simulink model "mcb_pmsm_fsfb_qep_f28379d"  (R2025b)
settings: Solver=FixedStepDiscrete  StartTime=0.0  StopTime=4  RelTol=1e-3  EnableMultiTasking=on
InitFcn:
  | mcb_pmsm_foc_qep_f28379d_SIUnit_data;
values from neighbouring files (symbols this model uses):
  A = [ -Rs/L,           0,                  0 ... (first row only)    [mcb_pmsm_fsfb_f28379d_param.m]    (also in v0_pmsm_fsfb_sim_for_flipsky_.m = [; v1_0_3_sim_param_fsfc.m = [)
  dataType = 'single'    [mcb_pmsm_foc_qep_f28379d_SIUnit_data.m]
  inverter = mcb.updateInverterParameters(pmsm,inverter,target)    [mcb_pmsm_foc_qep_f28379d_SIUnit_data.m]
  lambda_pm = pmsm.FluxPM    [mcb_pmsm_foc_qep_f28379d_SIUnit_data.m]
  PI_params = mcb.calcFOCGains(motor,Ts,Ts_speed,SpdLPFltCoeff=LPFltCoeff)    [mcb_pmsm_foc_qep_f28379d_SIUnit_data.m]
  pmsm = mcb.getPMSMParameters('Teknic2310P')    [mcb_pmsm_foc_qep_f28379d_SIUnit_data.m]
  T_pwm = 1/PWM_frequency    (= 5e-05)    [mcb_pmsm_foc_qep_f28379d_SIUnit_data.m]
  target = mcb.getProcessorParameters('F28379D',PWM_frequency)    [mcb_pmsm_foc_qep_f28379d_SIUnit_data.m]
  Ts = T_pwm    (= 5e-05)    [mcb_pmsm_foc_qep_f28379d_SIUnit_data.m]    (also in v0_pmsm_fsfb_sim_for_flipsky_.m = 0.0001; v1_0_3_sim_param_fsfc.m = 0.0001)
  Ts_inverter = T_pwm/2    (= 2.5e-05)    [mcb_pmsm_foc_qep_f28379d_SIUnit_data.m]
  Ts_motor = T_pwm/2    (= 2.5e-05)    [mcb_pmsm_foc_qep_f28379d_SIUnit_data.m]
  Ts_simulink = T_pwm/2    (= 2.5e-05)    [mcb_pmsm_foc_qep_f28379d_SIUnit_data.m]
  Ts_speed = 10*Ts    (= 0.0005)    [mcb_pmsm_foc_qep_f28379d_SIUnit_data.m]
undefined symbols (not defined in the file or in its folder): bit, DiscIntNeverNeededParam, Down, GPTRIP1SEL, GPTRIP2SEL, TZ1, TZ2, Up
libraries: mcbcontrolslib x8, c2802xlib x7, simulink x7, c280xlib x5, c2837xDlib x4, mcbeeMathTransformLib x3, slpidlib x3, mcbpositiondecoderlib x3, c2000lib x1, svdutilitieslib x1, autolibpmsmexterior x1
(part 1 of 2)
settings Model: ExtModeTrigDuration=8  Creator=The MathWorks, Inc.  LastModifiedBy=LabPC
settings SolverCC: AlgebraicLoopSolver=TrustRegion
settings OptimizationCC: DefaultParameterBehavior=Inlined  DefaultUnderspecifiedDataType=single  EnhancedBackFolding=on  PassReuseOutputArgsAs=Individual arguments  MaxStackSize=1024  OptimizeBlockOrder=speed  DifferentSizesBufferReuse=on  OptimizationCustomize=off  DenormalBehavior=FlushToZero  EfficientTunableParamExpr=on
settings DebuggingCC: MultiTaskDSMMsg=none  IntegerOverflowMsg=none  ParameterPrecisionLossMsg=none  ParameterTunabilityLossMsg=error  UnconnectedInputMsg=warning  UnconnectedOutputMsg=warning  UnconnectedLineMsg=warning
settings HardwareCC: ProdBitPerChar=16.0  ProdBitPerInt=16.0  ProdBitPerPointer=32.0  ProdBitPerSizeT=32.0  ProdBitPerPtrDiffT=32.0  ProdLargestAtomicInteger=Integer  ProdLargestAtomicFloat=None  ProdWordSize=16.0  ProdLongLongMode=on  ProdHWDeviceType=Texas Instruments->C2000
settings ModelReferenceCC: EnableRefExpFcnMdlSchedulingChecks=on
settings SFSimCC: MATLABDynamicMemAlloc=off
settings RTWCC: SystemTargetFile=ert.tlc  HardwareBoard=TI Delfino F28379D LaunchPad  TemplateMakefile=ert_default_tmf  Toolchain=Texas Instruments Code Composer Studio (C2000)  GPUComputeCapability=3.5  DLArmComputeVersion=19.05  Description=Embedded Coder
settings CodeAppCC: ForceParamTrailComments=on  IgnoreCustomStorageClasses=off  OperatorAnnotations=on  SimulinkDataObjDesc=on  SFDataObjDesc=on  InsertBlockDesc=on
settings ERTTargetCC: ExtModeStaticAllocSize=10000.0  InlinedParameterPlacement=Hierarchical  MemSecPackage=tic2000demospkg  DynamicArrayContainerType=coder::array  CodeReplacementLibrary=TI C28x

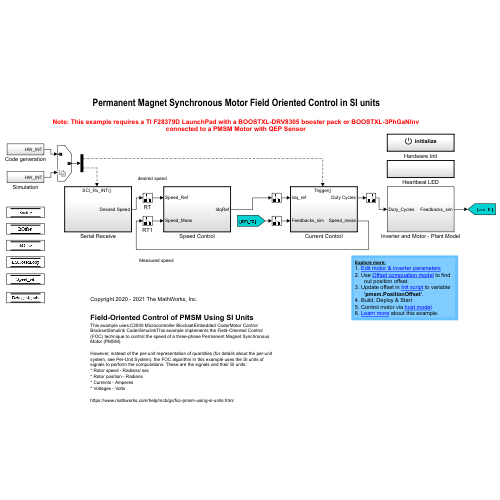
[thumbnail: Simulink's stored preview of the top-level diagram]
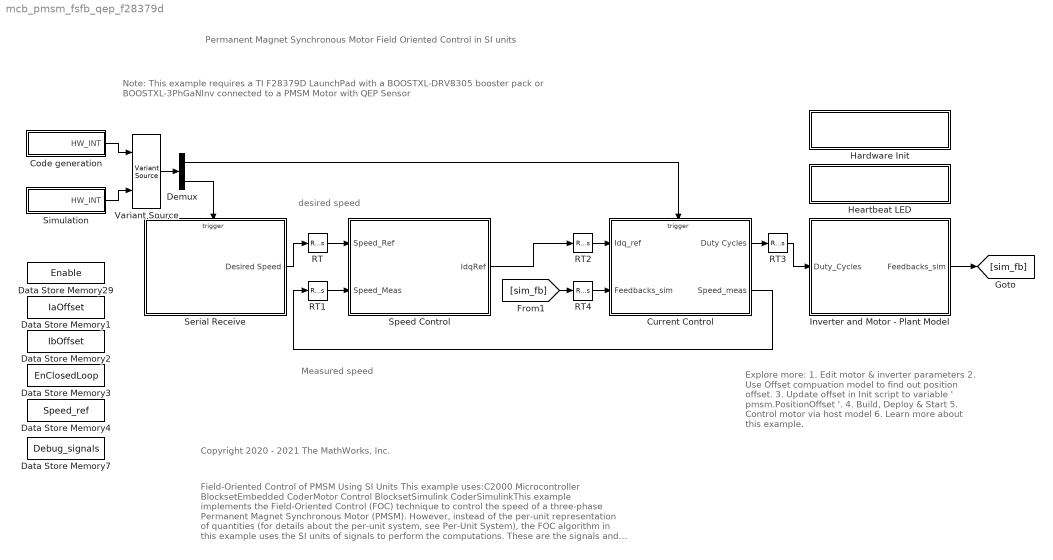
== system mcb_pmsm_fsfb_qep_f28379d ==
  note: Measured speed
  note: Field-Oriented Control of PMSM Using SI Units
      | This example uses:C2000 Microcontroller BlocksetEmbedded CoderMotor Control BlocksetSimulink CoderSimulinkThis example implements the Field-Oriented Control (FOC) technique to control the speed of a three-phase Permanent Magnet Synchronous Motor (PMSM).
      |
      | However, instead of the per-unit representation of quantities (for details about the per-unit system, see Per-Unit System), the FOC algorithm in this example uses the SI units of signals to perform the computations. These are the signals and their SI units:
      | * Rotor speed - Radians/ sec
      | * Rotor position - Radians
      | * Currents - Amperes
      | * Voltages - Volts
      |
      | https://www.mathworks.com/help/mcb/gs/foc-pmsm-using-si-units.html
  note: Permanent Magnet Synchronous Motor Field Oriented Control in SI units
  note: Copyright 2020 - 2021 The MathWorks, Inc.
  note: Note: This example requires a TI F28379D LaunchPad with a BOOSTXL-DRV8305 booster pack or BOOSTXL-3PhGaNInv
      | connected to a PMSM Motor with QEP Sensor
  note: Explore more:
      | 1. Edit motor & inverter parameters
      | 2. Use Offset compuation model to find out position offset.
      | 3. Update offset in Init script to variable ' pmsm.PositionOffset '.
      | 4. Build, Deploy & Start
      | 5. Control motor via host model
      | 6. Learn more about this example.
  note: desired speed
  Code generation : Subsystem
  Current Control : Subsystem
      settings: RTWSystemCode=Nonreusable function
  Data Store Memory1 : DataStoreMemory  DataStoreName=IaOffset  InitialValue=inverter.CtSensAOffset  ShowAdditionalParam=off
  Data Store Memory2 : DataStoreMemory  DataStoreName=IbOffset  InitialValue=inverter.CtSensBOffset  ShowAdditionalParam=off
  Data Store Memory29 : DataStoreMemory  DataStoreName=Enable  ShowAdditionalParam=off  OutDataTypeStr=boolean
  Data Store Memory3 : DataStoreMemory  DataStoreName=EnClosedLoop  ShowAdditionalParam=off  OutDataTypeStr=boolean
  Data Store Memory4 : DataStoreMemory  DataStoreName=Speed_ref  ShowAdditionalParam=off  OutDataTypeStr=dataType
  Data Store Memory7 : DataStoreMemory  DataStoreName=Debug_signals  InitialValue=5  ShowAdditionalParam=off  OutDataTypeStr=uint16
  Demux : Demux  Outputs=2
  Hardware Init : Subsystem  TreatAsAtomicUnit=on
  Heartbeat LED : Subsystem  TreatAsAtomicUnit=on
  Inverter and Motor - Plant Model : Subsystem
  RT : RateTransition  Deterministic=off  OutPortSampleTime=Ts_speed
  RT1 : RateTransition  Deterministic=off  OutPortSampleTime=Ts_speed
  RT2 : RateTransition  Deterministic=off
  RT3 : RateTransition  Deterministic=off
  RT4 : RateTransition  Deterministic=off
  Serial Receive : Subsystem  SystemSampleTime=1e-3
  Simulation : Subsystem
  Speed Control : Subsystem  TreatAsAtomicUnit=on  SystemSampleTime=Ts_speed
  Variant Source : VariantSource  VariantControlMode=sim codegen switching  VariantControls={(codegen), (sim)}
  wires:
  Speed Control/1(IdqRef) -> RT2/1
  Demux/2 -> Serial Receive/Trigger
  RT1/1 -> Speed Control/2(Speed_Meas)
  Serial Receive/1(Desired Speed) -> RT/1
  Code generation/1(HW_INT) -> Variant Source/1
  RT4/1 -> Current Control/2(Feedbacks_sim)
  Variant Source/1 -> Demux/1
  Current Control/1(Duty Cycles) -> RT3/1
  RT/1 -> Speed Control/1(Speed_Ref)
  Demux/1 -> Current Control/Trigger
  Simulation/1(HW_INT) -> Variant Source/2
  RT3/1 -> Inverter and Motor - Plant Model/1(Duty_Cycles)
  [sim_fb] -> RT4/1
  Current Control/2(Speed_meas) -> RT1/1
  Inverter and Motor - Plant Model/1(Feedbacks_sim) -> [sim_fb]
  RT2/1 -> Current Control/1(Idq_ref)

== system mcb_pmsm_fsfb_qep_f28379d/Code generation ==
  C28x Hardware Interrupt : c2000lib/Scheduling/C28x Hardware Interrupt  irqnumbers=[1 9]  pienumbers=[2 1]  irqpriorities=[30 50]  irqpreempts=[1 0]  showinput=off  dspchiptype=C280X
  HW_INT : Outport
  wires:
  C28x Hardware Interrupt/1 -> HW_INT/1

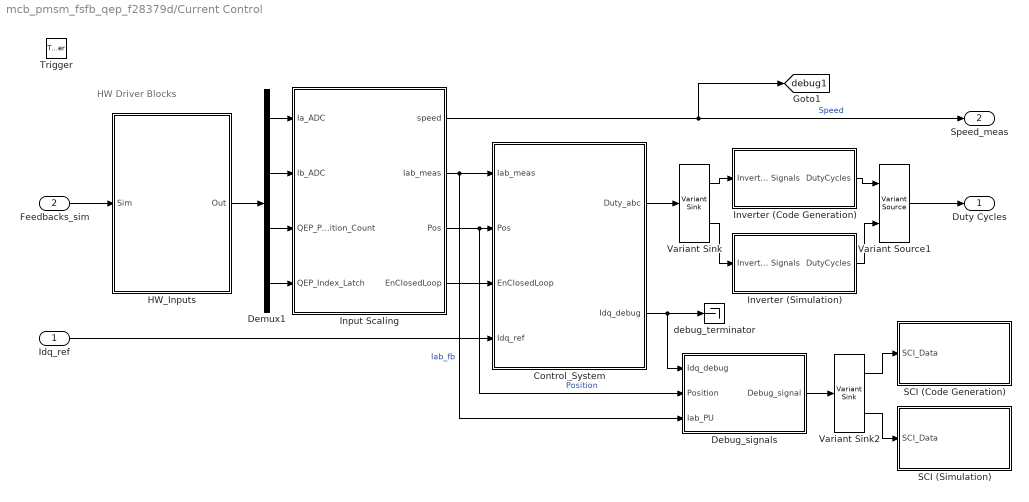
== system mcb_pmsm_fsfb_qep_f28379d/Current Control ==
  note: HW Driver Blocks
  Idq_ref : Inport
  Feedbacks_sim : Inport  Port=2
  Trigger : TriggerPort  TriggerType=function-call  VariantControl=Variant  PortDimensions=1
  Control_System : Subsystem  TreatAsAtomicUnit=on
  Debug_signals : Subsystem
  Demux1 : Demux
  HW_Inputs : Subsystem  Variant=on  VariantControlMode=sim codegen switching
  Input Scaling : Subsystem
  Inverter (Code Generation) : Subsystem
  Inverter (Simulation) : Subsystem
  SCI (Code Generation) : Subsystem
  SCI (Simulation) : Subsystem
  Variant Sink : VariantSink  VariantControlMode=sim codegen switching  VariantControls={(codegen), (sim)}
  Variant Sink2 : VariantSink  VariantControlMode=sim codegen switching  VariantControls={(codegen), (sim)}
  Variant Source1 : VariantSource  VariantControlMode=sim codegen switching  VariantControls={(codegen), (sim)}
  debug_terminator : Terminator
  Duty Cycles : Outport  InitialOutput=0  VectorParamsAs1DForOutWhenUnconnected=off
  Speed_meas : Outport  Port=2  InitialOutput=0  VectorParamsAs1DForOutWhenUnconnected=off
  tag scope: debug1=global
  wires:
  Control_System/1(Duty_abc) -> Variant Sink/1
  Input Scaling/3(Pos) -> Debug_signals/2(Position), Control_System/2(Pos)  "Position"
  Idq_ref/1 -> Control_System/4(Idq_ref)
  Input Scaling/1(speed) -> [debug1], Speed_meas/1  "Speed"
  Input Scaling/2(Iab_meas) -> Debug_signals/3(Iab_PU), Control_System/1(Iab_meas)  "Iab_fb"
  Demux1/1 -> Input Scaling/1(Ia_ADC)
  Demux1/2 -> Input Scaling/2(Ib_ADC)
  Demux1/3 -> Input Scaling/3(QEP_Position_Count)
  Demux1/4 -> Input Scaling/4(QEP_Index_Latch)
  Variant Sink2/1 -> SCI (Code Generation)/1(SCI_Data)
  Debug_signals/1(Debug_signal) -> Variant Sink2/1
  Inverter (Simulation)/1(DutyCycles) -> Variant Source1/2
  Inverter (Code Generation)/1(DutyCycles) -> Variant Source1/1
  Variant Sink2/2 -> SCI (Simulation)/1(SCI_Data)
  Variant Sink/2 -> Inverter (Simulation)/1(Inverter Signals)
  Variant Sink/1 -> Inverter (Code Generation)/1(Inverter Signals)
  Variant Source1/1 -> Duty Cycles/1
  HW_Inputs/1(Out) -> Demux1/1
  Feedbacks_sim/1 -> HW_Inputs/1(Sim)
  Control_System/2(Idq_debug) -> Debug_signals/1(Idq_debug), debug_terminator/1
  Input Scaling/4(EnClosedLoop) -> Control_System/3(EnClosedLoop)

== system mcb_pmsm_fsfb_qep_f28379d/Hardware Init ==
  6PWM_Mode : Constant  Priority=1000  Value=0x3A16  OutDataTypeStr=uint16  SampleTime=-1
  ADC_Gain_Setting : Constant  Priority=1000  Value=inverter.SPI_Gain_Setting  OutDataTypeStr=uint16  SampleTime=-1
  Code Generation : Subsystem
  Event Listener : EventListener  DisableCoverage=on  EventName=reset
  Mux : Mux  Inputs=2
  Simulation : Subsystem
  Variant Sink : VariantSink  VariantControlMode=sim codegen switching  VariantControls={(codegen), (sim)}
  wires:
  6PWM_Mode/1 -> Mux/1
  ADC_Gain_Setting/1 -> Mux/2
  Mux/1 -> Variant Sink/1
  Variant Sink/1 -> Code Generation/1(In)
  Variant Sink/2 -> Simulation/1(In1)

== system mcb_pmsm_fsfb_qep_f28379d/Heartbeat LED ==
  note: Heartbeat LED 1HZ
  Code generation : Subsystem
  RED_LED : Constant  OutDataTypeStr=uint16  SampleTime=0.5
  Simulation : Subsystem
  Variant Sink : VariantSink  VariantControlMode=sim codegen switching  VariantControls={(codegen), (sim)}
  wires:
  RED_LED/1 -> Variant Sink/1
  Variant Sink/1 -> Code generation/1(In1)
  Variant Sink/2 -> Simulation/1(In1)

== system mcb_pmsm_fsfb_qep_f28379d/Inverter and Motor - Plant Model ==
  Duty_Cycles : Inport
  Codegeneration : Subsystem
  Simulation : Subsystem
  Variant Sink : VariantSink  VariantControlMode=sim codegen switching  VariantControls={(codegen), (sim)}
  Variant Source1 : VariantSource  VariantControlMode=sim codegen switching  VariantControls={(codegen), (sim)}
  Feedbacks_sim : Outport  VectorParamsAs1DForOutWhenUnconnected=off
  wires:
  Variant Source1/1 -> Feedbacks_sim/1
  Simulation/1(Feedbacks) -> Variant Source1/2
  Codegeneration/1(Feedbacks) -> Variant Source1/1
  Duty_Cycles/1 -> Variant Sink/1
  Variant Sink/2 -> Simulation/1(Duty_Cycles)
  Variant Sink/1 -> Codegeneration/1(Duty_Cycles)

== system mcb_pmsm_fsfb_qep_f28379d/Serial Receive ==
  SCI_Rx_INT : TriggerPort  TriggerType=function-call  VariantControl=Variant
  Code Generation : Subsystem
  Data Store Write : DataStoreWrite  DataStoreName=Enable  IndexOptions=Index vector (dialog)  Indices=1  OutputSizes=1
  Data Store Write1 : DataStoreWrite  DataStoreName=Speed_ref  IndexOptions=Index vector (dialog)  Indices=1  OutputSizes=1
  Data Store Write2 : DataStoreWrite  DataStoreName=Debug_signals  IndexOptions=Index vector (dialog)  Indices=1  OutputSizes=1
  Data_Conditioning_Rx : Subsystem  Variant=on
  Simulation : Subsystem
  Variant Source : VariantSource  VariantControlMode=sim codegen switching  VariantControls={(codegen), (sim)}
  unParse : Subsystem
  Desired Speed : Outport  VectorParamsAs1DForOutWhenUnconnected=off
  wires:
  Simulation/1(Data) -> Variant Source/2
  Variant Source/1 -> Data_Conditioning_Rx/1(In1)
  Code Generation/1(Data) -> Variant Source/1
  unParse/1(Enable_PWM) -> Data Store Write/1
  Data_Conditioning_Rx/1(Desired Speed) -> Data Store Write1/1, Desired Speed/1
  Data_Conditioning_Rx/2(Out2) -> unParse/1(Data)
  unParse/2(Debug_signals) -> Data Store Write2/1

== system mcb_pmsm_fsfb_qep_f28379d/Simulation ==
  ADCINT1 : FunctionCallGenerator  SampleTime=Ts
  Mux : Mux  Inputs=2
  SCI_Rx_INT : FunctionCallGenerator  SampleTime=0.1
  HW_INT : Outport
  wires:
  SCI_Rx_INT/1 -> Mux/2
  ADCINT1/1 -> Mux/1
  Mux/1 -> HW_INT/1

== system mcb_pmsm_fsfb_qep_f28379d/Speed Control ==
  Speed_Ref : Inport
  Speed_Meas : Inport  Port=2
  Id_ref : Constant  Value=0  OutDataTypeStr=dataType  SampleTime=Ts_speed
  Mux1 : Mux  Inputs=2
  PI_Controller_Speed : Subsystem
  Subsystem : Subsystem
  IdqRef : Outport  VectorParamsAs1DForOutWhenUnconnected=off
  wires:
  Speed_Meas/1 -> PI_Controller_Speed/2(N_fb), Subsystem/2(Speed_Ref_Open)  "Speed_fb"
  Subsystem/1(Speed_Ref_PU) -> PI_Controller_Speed/1(N_ref)  "Speed_Ref"
  Id_ref/1 -> Mux1/1
  PI_Controller_Speed/1(Iq_ref) -> Mux1/2
  Mux1/1 -> IdqRef/1
  Speed_Ref/1 -> Subsystem/1(Speed_Ref_In)

== system mcb_pmsm_fsfb_qep_f28379d/Current Control/Control_System ==
  Iab_meas : Inport
  Pos : Inport  Port=2
  EnClosedLoop : Inport  Port=3
  Idq_ref : Inport  Port=4
  Closed Loop Control : Subsystem
  NOT : Logic  Operator=NOT  IconShape=distinctive  AllPortsSameDT=off  OutDataTypeStr=boolean
  Open Loop Start-Up : Subsystem
  Switch4 : Switch  Threshold=0.5  OutDataTypeStr=Inherit: Inherit via back propagation  RndMeth=Simplest  SaturateOnIntegerOverflow=off  InputSameDT=off
  Duty_abc : Outport  VectorParamsAs1DForOutWhenUnconnected=off
  Idq_debug : Outport  Port=2  VectorParamsAs1DForOutWhenUnconnected=off
  wires:
  EnClosedLoop/1 -> NOT/1, Switch4/2, Closed Loop Control/Enable
  Open Loop Start-Up/1(Duty_abc) -> Switch4/3
  Iab_meas/1 -> Closed Loop Control/1(Iab_meas)
  Pos/1 -> Closed Loop Control/2(Pos)
  Idq_ref/1 -> Closed Loop Control/3(Idq_ref)
  Closed Loop Control/2(Duty_abc) -> Switch4/1
  NOT/1 -> Open Loop Start-Up/Enable
  Switch4/1 -> Duty_abc/1  "PWM_Duty_Cycles"
  Closed Loop Control/1(Idq_debug) -> Idq_debug/1

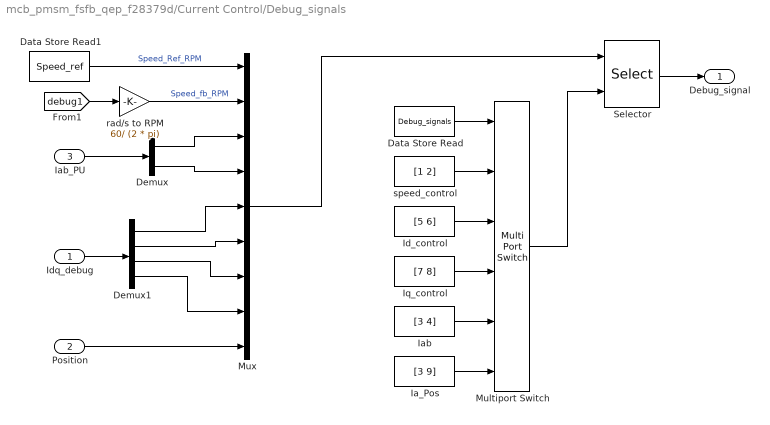
== system mcb_pmsm_fsfb_qep_f28379d/Current Control/Debug_signals ==
  Idq_debug : Inport
  Position : Inport  Port=2
  Iab_PU : Inport  Port=3
  Data Store Read : DataStoreRead  DataStoreName=Debug_signals  IndexOptions=Index vector (dialog)  Indices=1  OutputSizes=1
  Data Store Read1 : DataStoreRead  DataStoreName=Speed_ref  IndexOptions=Index vector (dialog)  Indices=1  OutputSizes=1
  Demux : Demux  Outputs=2
  Demux1 : Demux
  Ia_Pos : Constant  Value=[3 9]  OutDataTypeStr=uint16  SampleTime=-1
  Iab : Constant  Value=[3 4]  OutDataTypeStr=uint16  SampleTime=-1
  Id_control : Constant  Value=[5 6]  OutDataTypeStr=uint16  SampleTime=-1
  Iq_control : Constant  Value=[7 8]  OutDataTypeStr=uint16  SampleTime=-1
  Multiport Switch : MultiPortSwitch  Inputs=5  DiagnosticForDefault=Warning  OutDataTypeStr=uint16  RndMeth=Simplest  SaturateOnIntegerOverflow=off  InputSameDT=off
  Mux : Mux  Inputs=9
  Selector : Selector  InputPortWidth=9  IndexOptions=Index vector (port)  Indices=[1 3]  OutputSizes=1
  rad/s to RPM : Gain  Gain=60/ (2 * pi)  RndMeth=Simplest  OutDataTypeStr=Inherit: Same as input
  speed_control : Constant  Value=[1 2]  OutDataTypeStr=uint16  SampleTime=-1
  Debug_signal : Outport
  wires:
  speed_control/1 -> Multiport Switch/2
  Id_control/1 -> Multiport Switch/3
  Iq_control/1 -> Multiport Switch/4
  Iab/1 -> Multiport Switch/5
  Ia_Pos/1 -> Multiport Switch/6
  Multiport Switch/1 -> Selector/2
  Data Store Read/1 -> Multiport Switch/1
  Selector/1 -> Debug_signal/1
  Iab_PU/1 -> Demux/1
  Demux/1 -> Mux/3
  Demux/2 -> Mux/4
  Demux1/1 -> Mux/5
  Demux1/2 -> Mux/6
  Demux1/3 -> Mux/7
  Demux1/4 -> Mux/8
  Idq_debug/1 -> Demux1/1
  Mux/1 -> Selector/1
  Position/1 -> Mux/9
  [debug1] -> rad/s to RPM/1
  Data Store Read1/1 -> Mux/1  "Speed_Ref_RPM"
  rad/s to RPM/1 -> Mux/2  "Speed_fb_RPM"

== system mcb_pmsm_fsfb_qep_f28379d/Current Control/HW_Inputs ==
  Sim : Inport
  Sensor Driver Blocks (codegen) : Subsystem  VariantControl=(codegen)
  Sensor Driver Blocks (sim) : Subsystem  VariantControl=(sim)
  Out : Outport

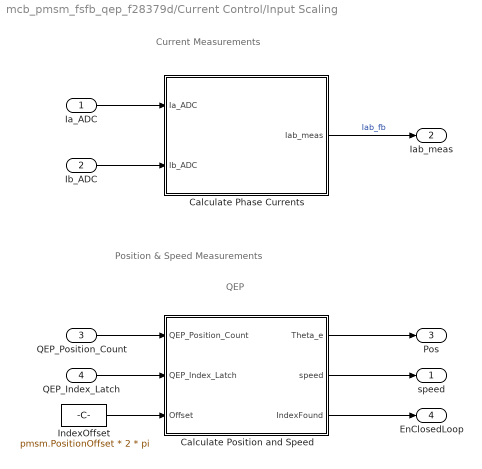
== system mcb_pmsm_fsfb_qep_f28379d/Current Control/Input Scaling ==
  note: Current Measurements
  note: Position & Speed Measurements
  note: QEP
  Ia_ADC : Inport
  Ib_ADC : Inport  Port=2
  QEP_Position_Count : Inport  Port=3
  QEP_Index_Latch : Inport  Port=4
  " Calculate Position and Speed" : Subsystem
  Calculate Phase Currents : Subsystem
  IndexOffset : Constant  Value=pmsm.PositionOffset * 2 * pi  OutDataTypeStr=dataType  SampleTime=-1
  speed : Outport
  Iab_meas : Outport  Port=2
  Pos : Outport  Port=3
  EnClosedLoop : Outport  Port=4
  wires:
  " Calculate Position and Speed"/2(speed) -> speed/1
  Calculate Phase Currents/1(Iab_meas) -> Iab_meas/1  "Iab_fb"
  QEP_Position_Count/1 -> " Calculate Position and Speed"/1(QEP_Position_Count)
  " Calculate Position and Speed"/1(Theta_e) -> Pos/1
  Ia_ADC/1 -> Calculate Phase Currents/1(Ia_ADC)
  Ib_ADC/1 -> Calculate Phase Currents/2(Ib_ADC)
  QEP_Index_Latch/1 -> " Calculate Position and Speed"/2(QEP_Index_Latch)
  IndexOffset/1 -> " Calculate Position and Speed"/3(Offset)
  " Calculate Position and Speed"/3(IndexFound) -> EnClosedLoop/1

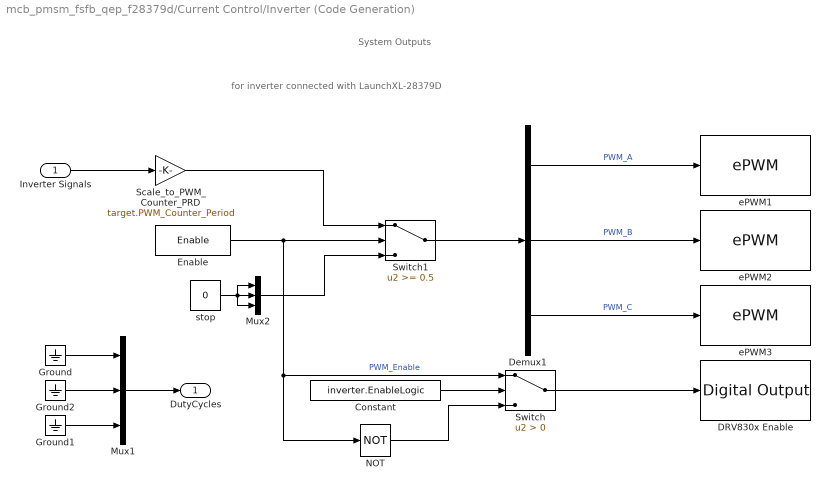
== system mcb_pmsm_fsfb_qep_f28379d/Current Control/Inverter (Code Generation) ==
  note: for inverter connected with LaunchXL-28379D
  note: System Outputs
  Inverter Signals : Inport
  Constant : Constant  Value=inverter.EnableLogic
  DRV830x Enable : c2837xDlib/Digital Output  GPIO_Number=GPIO120~GPIO127  GPIO_Bit0=off  GPIO_BIT0_Toggle=off  GPIO_Bit1=off  GPIO_BIT1_Toggle=off  GPIO_Bit2=off  GPIO_BIT2_Toggle=off  GPIO_Bit3=off  GPIO_BIT3_Toggle=off  GPIO_Bit4=on  GPIO_BIT4_Toggle=off  GPIO_Bit5=off  GPIO_BIT5_Toggle=off  GPIO_Bit6=off  GPIO_BIT6_Toggle=off  GPIO_Bit7=off  GPIO_BIT7_Toggle=off
  Demux1 : Demux  Outputs=3
  Enable : DataStoreRead  DataStoreName=Enable  IndexOptions=Index vector (dialog)  Indices=1  OutputSizes=1
  Ground : Ground
  Ground1 : Ground
  Ground2 : Ground
  Mux1 : Mux  Inputs=3
  Mux2 : Mux  Inputs=3
  NOT : Logic  Operator=NOT  IconShape=distinctive  AllPortsSameDT=off  OutDataTypeStr=boolean
  Scale_to_PWM_Counter_PRD : Gain  Gain=target.PWM_Counter_Period  OutDataTypeStr=uint16  RndMeth=Simplest
  Switch : Switch  Criteria=u2 > Threshold  SaturateOnIntegerOverflow=off  InputSameDT=off
  Switch1 : Switch  Threshold=0.5  SaturateOnIntegerOverflow=off  InputSameDT=off
  ePWM1 : c2802xlib/ePWM  PwmType=C2000_Type4  useModule=ePWM1  ePWMxLINKTBPRD=Not Linked  periodUnits=Clock cycles  timerSource=Specify via dialog  timerPeriod_clk=target.PWM_Counter_Period+1  timerPeriod_sec=0.0001  tbshadow=Counter equals to zero  countingMode=Up-Down  phaseActiveEnable=Disable  phaseDirection=Count down after sync  phaseActive=0  synchronizationEnable=off  dcaevt1Sync=off  dcbevt1Sync=off  synchronizationOption=Counter equals to zero (CTR=Zero)  dcbevt1SyncOut=off  dcaevt1SyncOut=off  cmpdSyncOut=off  cmpcSyncOut=off  cmpbSyncOut=off  zeroSyncOut=on  swfSyncOut=off  perSynchronizationOption=Counter equals to period (CTR=PRD)  clockPrescale=1  HSclockPrescale=1  enswap=off  ePWMxAStatus=on  ePWMxAactionLogic1=Do nothing  ePWMxAactionLogic2=Do nothing  ePWMxAactionLogic3=Clear  ePWMxAactionLogic4=Set  ePWMxAactionLogic5=Do nothing  ePWMxAactionLogic6=Do nothing  ePWMxACSFenable=off  ePWMxACSFvalue=Forcing disable  ePWMxASFreload=Zero  ePWMxBStatus=off  ePWMxBactionLogic1=Set  ePWMxBactionLogic2=Clear  ePWMxBactionLogic3=Do nothing  ePWMxBactionLogic4=Do nothing  ePWMxBactionLogic5=Clear  ePWMxBactionLogic6=Set  ePWMxBCSFenable=off  ePWMxBCSFvalue=Forcing disable  ePWMxBSFreload=Zero  ePWNxBOutWay=off  ePWMxLINKCMPA=Not Linked  CMPAUnits=Clock cycles  CMPASource=Input port  CMPAValue_per=50  CMPAValue_clk=floor(target.PWM_Counter_Period/2+1)  enCMPAshadow=Counter equals to zero (CTR=Zero)  ePWMxLINKCMPB=Not Linked  CMPBUnits=Clock cycles  CMPBSource=Specify via dialog  CMPBValue_per=50  CMPBValue_clk=floor(target.PWM_Counter_Period/2+1)  enCMPBshadow=Counter equals to zero (CTR=Zero)  ePWMxLINKCMPC=Not Linked  CMPCUnits=Clock cycles  CMPCSource=Specify via dialog  CMPCValue_per=50  CMPCValue_clk=32000  enCMPCshadow=Counter equals to zero (CTR=Zero)  ePWMxLINKCMPD=Not Linked  CMPDUnits=Clock cycles  CMPDSource=Specify via dialog  CMPDValue_per=50  CMPDValue_clk=32000  enCMPDshadow=Counter equals to zero (CTR=Zero)  enableDBePWMxA=on  enableDBePWMxB=on  enhalfcycle=off  DBpolarity=Active high complementary (AHC)  DBedgeDelay=Positive  DBSource_ePWMxA=ePWMxA  DBSource_ePWMxB=ePWMxA  DBPeriodUnits=Clock cycles  DBperiodSource=Specify via dialog  REDperiod=15  FEDperiod=15  REDperiod_sec=0  FEDperiod_sec=0  LoadModeDBRED=Immediate without using shadow  LoadModeDBFED=Immediate without using shadow  adcstartModuleA=on  adcrequestEventA=First event  adcstartEventA=Digital Compare Module A Event 1 start of conversion (DCAEVT1.soc)  adcstartEventA_type2=Counter equals to period (CTR=PRD)  adcstartModuleB=off  adcrequestEventB=First event  adcstartEventB=Counter equals to zero (CTR=Zero)  adcstartEventB_type2=Counter equals to zero (CTR=Zero)  intEn=off  intPrd=First event  intSel=Counter equals to zero (CTR=Zero)  intSel_type2=Counter equals to zero (CTR=Zero)  hrpe=off  enHRPWM=off  HRPWM_LoadMode=Counter equals to period (CTR=PRD)  HRPWM_CTLMode=Duty or Period control mode  HRPWM_EDGMode=Both edge  hrpeb=off  enHRPWMB=off  HRPWM_LoadModeB=Counter equals to zero (CTR=ZERO)  HRPWM_CTLModeB=Duty or Period control mode  HRPWM_EDGModeB=Both edge  enHRDBRED=off  enHRDBFED=off  enSFO=on  enautoconv=on  chopperEnable=off  chopperFrequency=1  chopperFirstwidth=1  chopperDuty=12.5%  tripZonesource=Specify via dialog  tzselOSHT1=off  tzselOSHT2=off  tzselOSHT3=off  tzselOSHT4=off  tzselOSHT5=off  tzselOSHT6=off  tzselOSHDCAEV1=off  tzselOSHDCBEV1=off  tzselCBC1=off  tzselCBC2=off  tzselCBC3=off  tzselCBC4=off  tzselCBC5=off  tzselCBC6=off  tzselCBCDCAEV2=off  tzselCBCDCBEV2=off  enTzOstIntr=off  enTzCbcIntr=off  enTzDCAEVT1Intr=off  enTzDCAEVT2Intr=off  enTzDCBEVT1Intr=off  enTzDCBEVT2Intr=off  tzclrCBCLatch=Counter equals to zero (CTR=Zero)  ePWMxAforced=No action  ePWMxBforced=No action  DCAEVT1forced=No action  DCBEVT1forced=No action  DCAEVT2forced=No action  DCBEVT2forced=No action  dcah=Trip Zone 1 input (TZ1)  dcal=Trip Zone 2 input (TZ2)  dcbh=Trip Zone 1 input (TZ1)  dcbl=Trip Zone 2 input (TZ2)  dcah_type2=GPTRIP1SEL/(TZ1)  dcal_type2=GPTRIP2SEL/(TZ2)  dcbh_type2=GPTRIP1SEL/(TZ1)  dcbl_type2=GPTRIP2SEL/(TZ2)  gendcaevt1=Event disabled  gendcaevt2=Event disabled  gendcbevt1=Event disabled  gendcbevt2=Event disabled  dcaevt1src=DCAEVT1 with sync  dcaevt2src=DCAEVT2 with sync  dcbevt1src=DCBEVT1 with sync  dcbevt2src=DCBEVT2 with sync  pulsesel=Counter equals to zero (CTR=Zero)  blankinv=off  blankoffset=0  blankwidth=0  evsrcsel=Filtered version of DCAEVT1 (DCAEVT1FILT)  encape=off
  ePWM2 : c2802xlib/ePWM  PwmType=C2000_Type4  useModule=ePWM2  ePWMxLINKTBPRD=Not Linked  periodUnits=Clock cycles  timerSource=Specify via dialog  timerPeriod_clk=target.PWM_Counter_Period+1  timerPeriod_sec=0.0001  tbshadow=Counter equals to zero  countingMode=Up-Down  phaseActiveEnable=Set counter to phase value specified via dialog  phaseDirection=Count up after sync  phaseActive=0  synchronizationEnable=off  dcaevt1Sync=off  dcbevt1Sync=off  synchronizationOption=Pass through (EPWMxSYNCI or SWFSYNC)  dcbevt1SyncOut=off  dcaevt1SyncOut=off  cmpdSyncOut=off  cmpcSyncOut=off  cmpbSyncOut=off  zeroSyncOut=off  swfSyncOut=on  perSynchronizationOption=Counter equals to period (CTR=PRD)  clockPrescale=1  HSclockPrescale=1  enswap=off  ePWMxAStatus=on  ePWMxAactionLogic1=Do nothing  ePWMxAactionLogic2=Do nothing  ePWMxAactionLogic3=Clear  ePWMxAactionLogic4=Set  ePWMxAactionLogic5=Do nothing  ePWMxAactionLogic6=Do nothing  ePWMxACSFenable=off  ePWMxACSFvalue=Forcing disable  ePWMxASFreload=Zero  ePWMxBStatus=off  ePWMxBactionLogic1=Set  ePWMxBactionLogic2=Clear  ePWMxBactionLogic3=Do nothing  ePWMxBactionLogic4=Do nothing  ePWMxBactionLogic5=Clear  ePWMxBactionLogic6=Set  ePWMxBCSFenable=off  ePWMxBCSFvalue=Forcing disable  ePWMxBSFreload=Zero  ePWNxBOutWay=off  ePWMxLINKCMPA=Not Linked  CMPAUnits=Clock cycles  CMPASource=Input port  CMPAValue_per=50  CMPAValue_clk=floor(target.PWM_Counter_Period/2+1)  enCMPAshadow=Counter equals to zero (CTR=Zero)  ePWMxLINKCMPB=Not Linked  CMPBUnits=Clock cycles  CMPBSource=Specify via dialog  CMPBValue_per=50  CMPBValue_clk=floor(target.PWM_Counter_Period/2+1)  enCMPBshadow=Counter equals to zero (CTR=Zero)  ePWMxLINKCMPC=Not Linked  CMPCUnits=Clock cycles  CMPCSource=Specify via dialog  CMPCValue_per=50  CMPCValue_clk=32000  enCMPCshadow=Counter equals to zero (CTR=Zero)  ePWMxLINKCMPD=Not Linked  CMPDUnits=Clock cycles  CMPDSource=Specify via dialog  CMPDValue_per=50  CMPDValue_clk=32000  enCMPDshadow=Counter equals to zero (CTR=Zero)  enableDBePWMxA=on  enableDBePWMxB=on  enhalfcycle=off  DBpolarity=Active high complementary (AHC)  DBedgeDelay=Positive  DBSource_ePWMxA=ePWMxA  DBSource_ePWMxB=ePWMxA  DBPeriodUnits=Clock cycles  DBperiodSource=Specify via dialog  REDperiod=15  FEDperiod=15  REDperiod_sec=0  FEDperiod_sec=0  LoadModeDBRED=Immediate without using shadow  LoadModeDBFED=Immediate without using shadow  adcstartModuleA=off  adcrequestEventA=First event  adcstartEventA=Digital Compare Module A Event 1 start of conversion (DCAEVT1.soc)  adcstartEventA_type2=Counter equals to period (CTR=PRD)  adcstartModuleB=off  adcrequestEventB=First event  adcstartEventB=Counter equals to zero (CTR=Zero)  adcstartEventB_type2=Counter equals to zero (CTR=Zero)  intEn=off  intPrd=First event  intSel=Counter equals to zero (CTR=Zero)  intSel_type2=Counter equals to zero (CTR=Zero)  hrpe=off  enHRPWM=off  HRPWM_LoadMode=Counter equals to period (CTR=PRD)  HRPWM_CTLMode=Duty or Period control mode  HRPWM_EDGMode=Both edge  hrpeb=off  enHRPWMB=off  HRPWM_LoadModeB=Counter equals to zero (CTR=ZERO)  HRPWM_CTLModeB=Duty or Period control mode  HRPWM_EDGModeB=Both edge  enHRDBRED=off  enHRDBFED=off  enSFO=on  enautoconv=on  chopperEnable=off  chopperFrequency=1  chopperFirstwidth=1  chopperDuty=12.5%  tripZonesource=Specify via dialog  tzselOSHT1=off  tzselOSHT2=off  tzselOSHT3=off  tzselOSHT4=off  tzselOSHT5=off  tzselOSHT6=off  tzselOSHDCAEV1=off  tzselOSHDCBEV1=off  tzselCBC1=off  tzselCBC2=off  tzselCBC3=off  tzselCBC4=off  tzselCBC5=off  tzselCBC6=off  tzselCBCDCAEV2=off  tzselCBCDCBEV2=off  enTzOstIntr=off  enTzCbcIntr=off  enTzDCAEVT1Intr=off  enTzDCAEVT2Intr=off  enTzDCBEVT1Intr=off  enTzDCBEVT2Intr=off  tzclrCBCLatch=Counter equals to zero (CTR=Zero)  ePWMxAforced=No action  ePWMxBforced=No action  DCAEVT1forced=No action  DCBEVT1forced=No action  DCAEVT2forced=No action  DCBEVT2forced=No action  dcah=Trip Zone 1 input (TZ1)  dcal=Trip Zone 2 input (TZ2)  dcbh=Trip Zone 1 input (TZ1)  dcbl=Trip Zone 2 input (TZ2)  dcah_type2=GPTRIP1SEL/(TZ1)  dcal_type2=GPTRIP2SEL/(TZ2)  dcbh_type2=GPTRIP1SEL/(TZ1)  dcbl_type2=GPTRIP2SEL/(TZ2)  gendcaevt1=Event disabled  gendcaevt2=Event disabled  gendcbevt1=Event disabled  gendcbevt2=Event disabled  dcaevt1src=DCAEVT1 with sync  dcaevt2src=DCAEVT2 with sync  dcbevt1src=DCBEVT1 with sync  dcbevt2src=DCBEVT2 with sync  pulsesel=Counter equals to zero (CTR=Zero)  blankinv=off  blankoffset=0  blankwidth=0  evsrcsel=Filtered version of DCAEVT1 (DCAEVT1FILT)  encape=off
  ePWM3 : c2802xlib/ePWM  PwmType=C2000_Type4  useModule=ePWM3  ePWMxLINKTBPRD=Not Linked  periodUnits=Clock cycles  timerSource=Specify via dialog  timerPeriod_clk=target.PWM_Counter_Period+1  timerPeriod_sec=0.0001  tbshadow=Counter equals to zero  countingMode=Up-Down  phaseActiveEnable=Set counter to phase value specified via dialog  phaseDirection=Count up after sync  phaseActive=0  synchronizationEnable=off  dcaevt1Sync=off  dcbevt1Sync=off  synchronizationOption=Pass through (EPWMxSYNCI or SWFSYNC)  dcbevt1SyncOut=off  dcaevt1SyncOut=off  cmpdSyncOut=off  cmpcSyncOut=off  cmpbSyncOut=off  zeroSyncOut=off  swfSyncOut=on  perSynchronizationOption=Counter equals to period (CTR=PRD)  clockPrescale=1  HSclockPrescale=1  enswap=off  ePWMxAStatus=on  ePWMxAactionLogic1=Do nothing  ePWMxAactionLogic2=Do nothing  ePWMxAactionLogic3=Clear  ePWMxAactionLogic4=Set  ePWMxAactionLogic5=Do nothing  ePWMxAactionLogic6=Do nothing  ePWMxACSFenable=off  ePWMxACSFvalue=Forcing disable  ePWMxASFreload=Zero  ePWMxBStatus=off  ePWMxBactionLogic1=Set  ePWMxBactionLogic2=Clear  ePWMxBactionLogic3=Do nothing  ePWMxBactionLogic4=Do nothing  ePWMxBactionLogic5=Clear  ePWMxBactionLogic6=Set  ePWMxBCSFenable=off  ePWMxBCSFvalue=Forcing disable  ePWMxBSFreload=Zero  ePWNxBOutWay=off  ePWMxLINKCMPA=Not Linked  CMPAUnits=Clock cycles  CMPASource=Input port  CMPAValue_per=50  CMPAValue_clk=floor(target.PWM_Counter_Period/2+1)  enCMPAshadow=Counter equals to zero (CTR=Zero)  ePWMxLINKCMPB=Not Linked  CMPBUnits=Clock cycles  CMPBSource=Specify via dialog  CMPBValue_per=50  CMPBValue_clk=floor(target.PWM_Counter_Period/2+1)  enCMPBshadow=Counter equals to zero (CTR=Zero)  ePWMxLINKCMPC=Not Linked  CMPCUnits=Clock cycles  CMPCSource=Specify via dialog  CMPCValue_per=50  CMPCValue_clk=32000  enCMPCshadow=Counter equals to zero (CTR=Zero)  ePWMxLINKCMPD=Not Linked  CMPDUnits=Clock cycles  CMPDSource=Specify via dialog  CMPDValue_per=50  CMPDValue_clk=32000  enCMPDshadow=Counter equals to zero (CTR=Zero)  enableDBePWMxA=on  enableDBePWMxB=on  enhalfcycle=off  DBpolarity=Active high complementary (AHC)  DBedgeDelay=Positive  DBSource_ePWMxA=ePWMxA  DBSource_ePWMxB=ePWMxA  DBPeriodUnits=Clock cycles  DBperiodSource=Specify via dialog  REDperiod=15  FEDperiod=15  REDperiod_sec=0  FEDperiod_sec=0  LoadModeDBRED=Immediate without using shadow  LoadModeDBFED=Immediate without using shadow  adcstartModuleA=off  adcrequestEventA=First event  adcstartEventA=Digital Compare Module A Event 1 start of conversion (DCAEVT1.soc)  adcstartEventA_type2=Counter equals to period (CTR=PRD)  adcstartModuleB=off  adcrequestEventB=First event  adcstartEventB=Counter equals to zero (CTR=Zero)  adcstartEventB_type2=Counter equals to zero (CTR=Zero)  intEn=off  intPrd=First event  intSel=Counter equals to zero (CTR=Zero)  intSel_type2=Counter equals to zero (CTR=Zero)  hrpe=off  enHRPWM=off  HRPWM_LoadMode=Counter equals to period (CTR=PRD)  HRPWM_CTLMode=Duty or Period control mode  HRPWM_EDGMode=Both edge  hrpeb=off  enHRPWMB=off  HRPWM_LoadModeB=Counter equals to zero (CTR=ZERO)  HRPWM_CTLModeB=Duty or Period control mode  HRPWM_EDGModeB=Both edge  enHRDBRED=off  enHRDBFED=off  enSFO=on  enautoconv=on  chopperEnable=off  chopperFrequency=1  chopperFirstwidth=1  chopperDuty=12.5%  tripZonesource=Specify via dialog  tzselOSHT1=off  tzselOSHT2=off  tzselOSHT3=off  tzselOSHT4=off  tzselOSHT5=off  tzselOSHT6=off  tzselOSHDCAEV1=off  tzselOSHDCBEV1=off  tzselCBC1=off  tzselCBC2=off  tzselCBC3=off  tzselCBC4=off  tzselCBC5=off  tzselCBC6=off  tzselCBCDCAEV2=off  tzselCBCDCBEV2=off  enTzOstIntr=off  enTzCbcIntr=off  enTzDCAEVT1Intr=off  enTzDCAEVT2Intr=off  enTzDCBEVT1Intr=off  enTzDCBEVT2Intr=off  tzclrCBCLatch=Counter equals to zero (CTR=Zero)  ePWMxAforced=No action  ePWMxBforced=No action  DCAEVT1forced=No action  DCBEVT1forced=No action  DCAEVT2forced=No action  DCBEVT2forced=No action  dcah=Trip Zone 1 input (TZ1)  dcal=Trip Zone 2 input (TZ2)  dcbh=Trip Zone 1 input (TZ1)  dcbl=Trip Zone 2 input (TZ2)  dcah_type2=GPTRIP1SEL/(TZ1)  dcal_type2=GPTRIP2SEL/(TZ2)  dcbh_type2=GPTRIP1SEL/(TZ1)  dcbl_type2=GPTRIP2SEL/(TZ2)  gendcaevt1=Event disabled  gendcaevt2=Event disabled  gendcbevt1=Event disabled  gendcbevt2=Event disabled  dcaevt1src=DCAEVT1 with sync  dcaevt2src=DCAEVT2 with sync  dcbevt1src=DCBEVT1 with sync  dcbevt2src=DCBEVT2 with sync  pulsesel=Counter equals to zero (CTR=Zero)  blankinv=off  blankoffset=0  blankwidth=0  evsrcsel=Filtered version of DCAEVT1 (DCAEVT1FILT)  encape=off
  stop : Constant  Value=0  OutDataTypeStr=uint16
  DutyCycles : Outport  VectorParamsAs1DForOutWhenUnconnected=off
  wires:
  Demux1/3 -> ePWM3/1  "PWM_C"
  Scale_to_PWM_Counter_PRD/1 -> Switch1/1
  Mux2/1 -> Switch1/3
  stop/1 -> Mux2/3, Mux2/2, Mux2/1
  Enable/1 -> Switch/1, NOT/1, Switch1/2  "PWM_Enable"
  Demux1/2 -> ePWM2/1  "PWM_B"
  Switch1/1 -> Demux1/1
  Demux1/1 -> ePWM1/1  "PWM_A"
  Inverter Signals/1 -> Scale_to_PWM_Counter_PRD/1
  Ground/1 -> Mux1/1
  Ground1/1 -> Mux1/3
  Ground2/1 -> Mux1/2
  Mux1/1 -> DutyCycles/1
  Switch/1 -> DRV830x Enable/1
  NOT/1 -> Switch/3
  Constant/1 -> Switch/2

== system mcb_pmsm_fsfb_qep_f28379d/Current Control/Inverter (Simulation) ==
  Inverter Signals : Inport
  Data Type Duplicate : DataTypeDuplicate
  Enable : DataStoreRead  DataStoreName=Enable  IndexOptions=Index vector (dialog)  Indices=1  OutputSizes=1
  Mux2 : Mux  Inputs=3
  Switch1 : Switch  Threshold=0.5  RndMeth=Simplest  SaturateOnIntegerOverflow=off  InputSameDT=off
  stop : Constant  Value=0  OutDataTypeStr=Inherit: Inherit via back propagation
  DutyCycles : Outport  VectorParamsAs1DForOutWhenUnconnected=off
  wires:
  stop/1 -> Data Type Duplicate/2, Mux2/1, Mux2/3, Mux2/2
  Mux2/1 -> Switch1/3
  Switch1/1 -> DutyCycles/1
  Inverter Signals/1 -> Data Type Duplicate/1, Switch1/1  "PWM Duty Cycles"
  Enable/1 -> Switch1/2  "PWM_Enable"

== system mcb_pmsm_fsfb_qep_f28379d/Current Control/SCI (Code Generation) ==
  SCI_Data : Inport
  Data_Conditioning_Tx : Subsystem  Variant=on
  Data_Logging : Subsystem
  Demux2 : Demux  Outputs=2
  While Iterator Subsystem : Subsystem  TreatAsAtomicUnit=on
  wires:
  Demux2/2 -> While Iterator Subsystem/2(Iteration)  "SCI_Tx_Iteration"
  Demux2/1 -> While Iterator Subsystem/1(Data)  "SCI_Tx_Data"
  SCI_Data/1 -> Data_Conditioning_Tx/1(In1)
  Data_Logging/1(SCI_Tx) -> Demux2/1
  Data_Conditioning_Tx/1(Data_Log) -> Data_Logging/1(Data_Log)

== system mcb_pmsm_fsfb_qep_f28379d/Current Control/SCI (Simulation) ==
  SCI_Data : Inport
  Demux : Demux  Outputs=2
  Terminator1 : Terminator
  Terminator2 : Terminator
  wires:
  SCI_Data/1 -> Demux/1
  Demux/1 -> Terminator1/1
  Demux/2 -> Terminator2/1

== system mcb_pmsm_fsfb_qep_f28379d/Hardware Init/Code Generation ==
  note: for BoostXL-DRV8305 connected to LaunchXL-28379D
  note: System Outputs
  note: Enable ADC offset calibration only when motor is not loaded and not rotating due to external factors
  In : Inport
  ADC Calibration Enable : Constant  Value=inverter.ADCOffsetCalibEnable
  "Calculate ADC Offset " : Subsystem  Priority=1001  TreatAsAtomicUnit=on
  DRV Enable : Subsystem  Priority=1
  Default ADC Offset : Subsystem  Priority=1001  TreatAsAtomicUnit=on
  NOT : Logic  Operator=NOT  IconShape=distinctive  AllPortsSameDT=off  OutDataTypeStr=boolean
  wires:
  In/1 -> DRV Enable/1(In)
  NOT/1 -> Default ADC Offset/Enable
  ADC Calibration Enable/1 -> NOT/1, "Calculate ADC Offset "/Enable

== system mcb_pmsm_fsfb_qep_f28379d/Hardware Init/Simulation ==
  In1 : Inport
  Terminator : Terminator
  wires:
  In1/1 -> Terminator/1

== system mcb_pmsm_fsfb_qep_f28379d/Heartbeat LED/Code generation ==
  In1 : Inport
  Digital Output : c2837xDlib/Digital Output  GPIO_Number=GPIO32~GPIO39  GPIO_Bit0=off  GPIO_BIT0_Toggle=on  GPIO_Bit1=off  GPIO_BIT1_Toggle=off  GPIO_Bit2=on  GPIO_BIT2_Toggle=on  GPIO_Bit3=off  GPIO_BIT3_Toggle=off  GPIO_Bit4=off  GPIO_BIT4_Toggle=off  GPIO_Bit5=off  GPIO_BIT5_Toggle=off  GPIO_Bit6=off  GPIO_BIT6_Toggle=off  GPIO_Bit7=off  GPIO_BIT7_Toggle=off
  wires:
  In1/1 -> Digital Output/1

== system mcb_pmsm_fsfb_qep_f28379d/Heartbeat LED/Simulation ==
  In1 : Inport
  Simulation_Terminator : Terminator
  wires:
  In1/1 -> Simulation_Terminator/1

== system mcb_pmsm_fsfb_qep_f28379d/Inverter and Motor - Plant Model/Codegeneration ==
  Duty_Cycles : Inport
  Ground : Ground
  Terminator : Terminator
  Feedbacks : Outport  VectorParamsAs1DForOutWhenUnconnected=off
  wires:
  Duty_Cycles/1 -> Terminator/1
  Ground/1 -> Feedbacks/1

== system mcb_pmsm_fsfb_qep_f28379d/Inverter and Motor - Plant Model/Simulation ==
  Duty_Cycles : Inport
  Inverter : Subsystem
  Load_Profile (Torque) : Subsystem
  RT1 : RateTransition  Deterministic=off  OutPortSampleTime=Ts_simulink
  RT3 : RateTransition  Deterministic=off  OutPortSampleTime=Ts_simulink
  Rate Transition : RateTransition  Integrity=off  OutPortSampleTime=Ts_motor
  Rate Transition1 : RateTransition  Integrity=off  OutPortSampleTime=Ts_motor
  Sensor_Measurements : Subsystem
  Surface Mount PMSM : autolibpmsmexterior/Surface Mount PMSM  port_config=Torque  sim_type=Discrete  Ts=Ts_motor  P=pmsm.p  Rs=pmsm.Rs + inverter.R_board  Ldq_=pmsm.Ld  KConstText=Permanent flux linkage constant (lambda_pm):  lambda_pm=pmsm.FluxPM  Ke=159.9771  Kt=1.323  mechanical=[pmsm.J, pmsm.B, 0]  idq0=[0 0]  theta_init=0  omega_init=0  KConst=pmsm.FluxPM  lambda_pm_calc=pmsm.FluxPM  RefBlkName='autolibpmsmexterior/Surface Mount PMSM'  aMode=5  Ldq="[0.00105     0.00105]"
  Terminator : Terminator
  Feedbacks : Outport  VectorParamsAs1DForOutWhenUnconnected=off
  wires:
  Rate Transition1/1 -> Surface Mount PMSM/1
  Surface Mount PMSM/2 -> RT1/1  "Iabc"
  Surface Mount PMSM/3 -> Terminator/1
  Rate Transition/1 -> Surface Mount PMSM/2  "PhaseVoltage"
  RT1/1 -> Sensor_Measurements/2(PhaseCurr)
  Duty_Cycles/1 -> Inverter/1(Duty_abc)
  Inverter/1(Vabc) -> Rate Transition/1
  RT3/1 -> Sensor_Measurements/1(Info)
  Surface Mount PMSM/1 -> RT3/1
  Load_Profile (Torque)/1(Load_Trq) -> Rate Transition1/1
  Sensor_Measurements/1(Sim_fb) -> Feedbacks/1

== system mcb_pmsm_fsfb_qep_f28379d/Serial Receive/Code Generation ==
  SCI Receive : c280xlib/SCI Receive  sciModule=A  dataHead=''  headerCheckMaxCount=16  dataTail=''  dataType=single  dataLenOptions=Length via dialog  dataDim=2  maxDataLength=1  initValue=0  errOption=Output the last received value  errValue=0  sampleTime=-1  blockingMode=on  timeOut=0.00875  outputStatus=off
  Data : Outport
  wires:
  SCI Receive/1 -> Data/1

== system mcb_pmsm_fsfb_qep_f28379d/Serial Receive/Data_Conditioning_Rx ==
  In1 : Inport
  Data_Type_Fixed_Point : Subsystem  VariantControl=~isequal(dataType, 'single')
  Data_Type_Float : Subsystem  VariantControl=isequal(dataType, 'single')
  Desired Speed : Outport
  Out2 : Outport  Port=2

== system mcb_pmsm_fsfb_qep_f28379d/Serial Receive/Simulation ==
  Data Type Conversion2 : DataTypeConversion  OutDataTypeStr=dataType  RndMeth=Simplest  SaturateOnIntegerOverflow=off
  Data_Conditioning_Tx : Subsystem  Variant=on
  Debug_signals : Constant  OutDataTypeStr=uint16  SampleTime=-1
  Enable : Constant  OutDataTypeStr=uint16  SampleTime=-1
  Parse : Subsystem
  Reversal : Step  Time=3
  Speed_Ref_Final (rpm) : Constant  Value=-4000  OutDataTypeStr=double  SampleTime=-1
  Speed_Ref_Init (rpm) : Step  Before=1200  After=4000
  Switch : Switch  Criteria=u2 > Threshold  SaturateOnIntegerOverflow=off  InputSameDT=off
  Data : Outport
  wires:
  Data_Conditioning_Tx/1(Data) -> Data/1
  Speed_Ref_Final (rpm)/1 -> Switch/1
  Speed_Ref_Init (rpm)/1 -> Switch/3
  Reversal/1 -> Switch/2
  Enable/1 -> Parse/1(Enable_PWM)
  Debug_signals/1 -> Parse/2(Debug_signals)
  Parse/1(Data) -> Data_Conditioning_Tx/2(In2)
  Switch/1 -> Data Type Conversion2/1
  Data Type Conversion2/1 -> Data_Conditioning_Tx/1(In1)

== system mcb_pmsm_fsfb_qep_f28379d/Serial Receive/unParse ==
  Data : Inport
  Bitwise Operator : simulink/Logic and Bit Operations/Bitwise Operator  logicop=AND  UseBitMask=on  BitMask=hex2dec('0001')  BitMaskRealWorld=Stored Integer
  Bitwise Operator1 : simulink/Logic and Bit Operations/Bitwise Operator  logicop=AND  UseBitMask=on  BitMask=hex2dec('00F0')  BitMaskRealWorld=Stored Integer
  Data Type Conversion3 : DataTypeConversion  OutDataTypeStr=boolean  RndMeth=Simplest  SaturateOnIntegerOverflow=off
  Data Type Conversion4 : DataTypeConversion  OutDataTypeStr=uint16  RndMeth=Simplest  SaturateOnIntegerOverflow=off
  Shift Arithmetic1 : ArithShift  BitShiftNumber=4
  Enable_PWM : Outport
  Debug_signals : Outport  Port=2
  wires:
  Bitwise Operator1/1 -> Shift Arithmetic1/1
  Data/1 -> Bitwise Operator/1, Bitwise Operator1/1
  Bitwise Operator/1 -> Data Type Conversion3/1
  Data Type Conversion4/1 -> Debug_signals/1
  Shift Arithmetic1/1 -> Data Type Conversion4/1
  Data Type Conversion3/1 -> Enable_PWM/1

== system mcb_pmsm_fsfb_qep_f28379d/Speed Control/PI_Controller_Speed ==
  N_ref : Inport
  N_fb : Inport  Port=2
  Data Store Read1 : DataStoreRead  DataStoreName=Enable  IndexOptions=Index vector (dialog)  Indices=1  OutputSizes=1
  Discrete PI Controller with anti-windup & reset : slpidlib/PID Controller  Controller=PI  Form=Parallel  TimeDomain=Discrete-time  UseExternalTs=off  SampleTime=-1  IntegratorMethod=Forward Euler  FilterMethod=Forward Euler  ControllerParametersSource=external  P=1  I=1  UseKiTs=on  D=0  UseExternalDerivativeSource=off  N=100  UseFilter=on  TunerSelectOption=Transfer Function Based (PID Tuner App)  InitialConditionSource=external  InitialConditionForIntegrator=0  InitialConditionForFilter=0  DifferentiatorICPrevScaledInput=0  ExternalReset=level  TrackingMode=off  Kt=1  LimitOutput=on  SatLimitsSource=internal  UpperSaturationLimit=inverter.ISenseMax  LowerSaturationLimit=-inverter.ISenseMax  LinearizeAsGain=on  AntiWindupMode=clamping  Kb=1  LimitIntegrator=off  UpperIntegratorSaturationLimit=inf  LowerIntegratorSaturationLimit=-inf  RndMeth=Simplest  POutMin=[]  POutMax=[]  IOutMin=[]  IOutMax=[]  DOutMin=[]  DOutMax=[]  NOutMin=[]  NOutMax=[]  SumOutMin=[]  SumOutMax=[]  SaturationOutDataTypeStr=Inherit: Inherit via back propagation  SaturationOutMin=[]  SaturationOutMax=[]  PParamMin=[]  PParamMax=[]  IParamMin=[]  IParamMax=[]  DParamMin=[]  DParamMax=[]  NParamMin=[]  NParamMax=[]  KbParamMin=[]  KbParamMax=[]  KtParamMin=[]  KtParamMax=[]  KbOutMin=[]  KbOutMax=[]  KtOutMin=[]  KtOutMax=[]  IntegratorOutMin=[]  IntegratorOutMax=[]  FilterOutMin=[]  FilterOutMax=[]  SumI1OutMin=[]  SumI1OutMax=[]  SumI2OutMin=[]  SumI2OutMax=[]  SumI3OutMin=[]  SumI3OutMax=[]  SumI4OutMin=[]  SumI4OutMax=[]  SumDOutMin=[]  SumDOutMax=[]  DifferentiatorOutMin=[]  DifferentiatorOutMax=[]  FilterDiffOutCoefMin=[]  FilterDiffOutCoefMax=[]  ReciprocalOutMin=[]  ReciprocalOutMax=[]  SumDenOutMin=[]  SumDenOutMax=[]  SumNumOutMin=[]  SumNumOutMax=[]  DivideOutMin=[]  DivideOutMax=[]  UdiffTsProdOutMin=[]  UdiffTsProdOutMax=[]  NTsProdOutMin=[]  NTsProdOutMax=[]  UintegralTsProdOutMin=[]  UintegralTsProdOutMax=[]  UngainTsProdOutMin=[]  UngainTsProdOutMax=[]  ClampingZeroOutDataTypeStr=Inherit: Inherit via back propagation  ClampingZeroOutMin=[]  ClampingZeroOutMax=[]  FilterDenConstantOutDataTypeStr=Inherit: Inherit via back propagation  FilterDenConstantOutMin=[]  FilterDenConstantOutMax=[]  PCopyOutDataTypeStr=Inherit: Inherit via back propagation  PCopyOutMin=[]  PCopyOutMax=[]  NCopyOutDataTypeStr=Inherit: Inherit via back propagation  NCopyOutMin=[]  NCopyOutMax=[]  IntegratorContinuousStateAttributes=''  IntegratorStateMustResolveToSignalObject=off  IntegratorRTWStateStorageClass=Auto  FilterContinuousStateAttributes=''  FilterStateMustResolveToSignalObject=off  FilterRTWStateStorageClass=Auto  ParallelPVariant=ExternalParameters  IdealPVariant=Disabled  IVariant=ExternalParameters  DVariant=Disabled  IntegratorVariant=Discrete  SatVariant=Enabled  AWVariant=DiscClampingParallel  PCopyVariant=Disabled  TRVariant=Disabled  FdbkBlocksVariant=Forward  IdealPFdbkVariant=Disabled  SatFdbkVariant=Disabled  DerivativeFilterVariant=Disabled  NVariant=Disabled  NCopyVariant=Disabled_SignalSpec  FilterICVariant=Disabled  IntegratorICVariant=ExternalICs  ExternalResetVariant=ExternalReset  TRSumVariant=Passthrough  SumFdbkVariant=Disabled  SumVariant=Sum_PI  TsampFilterVariant=InternalTs  TsampNgainVariant=Passthrough  TsampIntegralVariant=Disabled_SignalSpec  ExternalSaturationOutDataTypeStr=Inherit: Same as second input  DerivativeSourceVariant=Disabled  PreIntVariant=InternalPreInt
      settings: LibrarySourceBlock=mcbcontrolslib/PI Controller
  Ki1 : Constant  Value=PI_params.Ki_speed * Ts_speed * inverter.ISenseMax  OutDataTypeStr=dataType  SampleTime=-1
  Ki2 : Constant  Value=0  OutDataTypeStr=dataType  SampleTime=-1
  Kp1 : Constant  Value=PI_params .Kp_speed * inverter.ISenseMax  OutDataTypeStr=dataType  SampleTime=-1
  Logical Operator : Logic  Operator=NOT  IconShape=distinctive  AllPortsSameDT=off  OutDataTypeStr=boolean
  Sum : Sum  Inputs=|+-  OutDataTypeStr=Inherit: Same as first input
  Zero_Cancellation : mcbcontrolslib/IIR Filter  VariantControl=Low Pass Filter  VariantSelect=Low-pass  FilterConstantInputType=Specify via dialog  Filter_constant=0.01*(Ts_speed/Ts)  InitialOutput=Specify via dialog  InitialOutputValue=0  ExternalReset=none  advancedSettings=off  Ts=50e-6  cutOff_freq=1
  Iq_ref : Outport  VectorParamsAs1DForOutWhenUnconnected=off
  wires:
  Discrete PI Controller with anti-windup & reset/1 -> Iq_ref/1
  Ki1/1 -> Discrete PI Controller with anti-windup & reset/3
  Kp1/1 -> Discrete PI Controller with anti-windup & reset/2
  Sum/1 -> Discrete PI Controller with anti-windup & reset/1
  Logical Operator/1 -> Discrete PI Controller with anti-windup & reset/4
  Ki2/1 -> Discrete PI Controller with anti-windup & reset/5
  Data Store Read1/1 -> Logical Operator/1
  N_ref/1 -> Zero_Cancellation/1
  N_fb/1 -> Sum/2
  Zero_Cancellation/1 -> Sum/1

== system mcb_pmsm_fsfb_qep_f28379d/Speed Control/Subsystem ==
  Speed_Ref_In : Inport
  Speed_Ref_Open : Inport  Port=2
  AND : Logic  IconShape=distinctive  AllPortsSameDT=off  OutDataTypeStr=boolean
  Data Store Read : DataStoreRead  DataStoreName=EnClosedLoop  IndexOptions=Index vector (dialog)  Indices=1  OutputSizes=1
  Data Store Read1 : DataStoreRead  DataStoreName=Enable  IndexOptions=Index vector (dialog)  Indices=1  OutputSizes=1
  RPM to rad/s : Gain  Gain=2 * pi / 60  RndMeth=Simplest  OutDataTypeStr=Inherit: Same as input
  Switch : Switch  Criteria=u2 > Threshold  Threshold=0.5  SaturateOnIntegerOverflow=off  InputSameDT=off
  Speed_Ref_PU : Outport
  wires:
  Switch/1 -> Speed_Ref_PU/1
  Speed_Ref_Open/1 -> Switch/3
  AND/1 -> Switch/2
  Data Store Read/1 -> AND/1
  Data Store Read1/1 -> AND/2
  Speed_Ref_In/1 -> RPM to rad/s/1
  RPM to rad/s/1 -> Switch/1

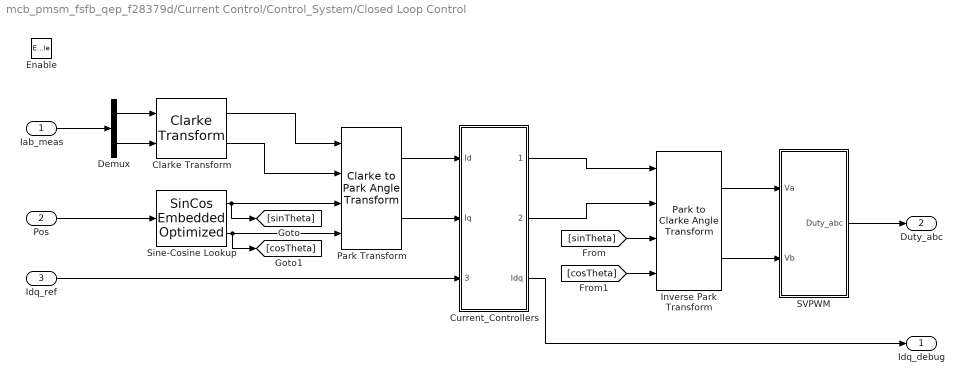
== system mcb_pmsm_fsfb_qep_f28379d/Current Control/Control_System/Closed Loop Control ==
  Iab_meas : Inport
  Pos : Inport  Port=2
  Idq_ref : Inport  Port=3
  Enable : EnablePort  StatesWhenEnabling=reset
  Clarke Transform : mcbeeMathTransformLib/Clarke Transform  VariantControl=Variant2  PowerInvariant=off  UseWithEmbedded=on  PhaseInput=Two inputs
  Current_Controllers : Subsystem
  Demux : Demux  Outputs=2
  Inverse Park Transform : mcbeeMathTransformLib/Park to Clarke Angle Transform  AxisAlignment=D-axis  UseWithEmbedded=on  PhaseInput=Two inputs  ThetaInput=Sine and Cosine electrical position  AngleInput=Per-unit  N_points=1024
  Park Transform : mcbeeMathTransformLib/Clarke to Park Angle Transform  AxisAlignment=D-axis  UseWithEmbedded=on  PhaseInput=Two inputs  ThetaInput=Sine and Cosine electrical position  AngleInput=Per-unit  N_points=1024
  SVPWM : Subsystem
  Sine-Cosine Lookup : mcbcontrolslib/SinCos Embedded Optimized  LabelModeActiveChoice=MCB_Sin  OptforProc=off  ApproximationMethod=None  UserApproxMethod=Lookup  ApproxStatus=None  InterpMethod=Linear point-slope  NumberOfDataPoints=16  NumberOfIterations=11  RemoveProtectionAgainstOutOfRangeInput=off  TableDataTypeStr=Inherit: Inherit via input  AngleInput=Radians  ThetaDataType=single  N_points=1024  DatatypeInput=Inherit from input  Datatype=Inherit: Same as input
  Idq_debug : Outport  VectorParamsAs1DForOutWhenUnconnected=off
  Duty_abc : Outport  Port=2  VectorParamsAs1DForOutWhenUnconnected=off
  wires:
  Iab_meas/1 -> Demux/1
  Park Transform/2 -> Current_Controllers/2(Iq)
  Park Transform/1 -> Current_Controllers/1(Id)
  Sine-Cosine Lookup/2 -> Park Transform/4, [cosTheta]
  Clarke Transform/1 -> Park Transform/1
  Idq_ref/1 -> Current_Controllers/3(Ida_ref)
  Sine-Cosine Lookup/1 -> [sinTheta], Park Transform/3
  Clarke Transform/2 -> Park Transform/2
  [cosTheta] -> Inverse Park Transform/4
  Demux/2 -> Clarke Transform/2
  Pos/1 -> Sine-Cosine Lookup/1
  Demux/1 -> Clarke Transform/1
  [sinTheta] -> Inverse Park Transform/3
  Current_Controllers/1(Vd_ref) -> Inverse Park Transform/1
  Current_Controllers/2(Vq_ref) -> Inverse Park Transform/2
  Current_Controllers/3(Idq) -> Idq_debug/1
  Inverse Park Transform/1 -> SVPWM/1(Va)
  Inverse Park Transform/2 -> SVPWM/2(Vb)
  SVPWM/1(Duty_abc) -> Duty_abc/1
